simulink model "ferreira_charlton"  (R2024b)
settings: Solver=ode4  StartTime=0.0  StopTime=20  FixedStep=2e-4  RelTol=1e-3
InitFcn:
  | parameters_charlton;
  | parameters_ferreira;
  | KT = 1.44; Tmax = KT*Tmax;
  | Emax = 1.4;
  | LAP = 8.50;
undefined symbols (not defined in the file): AP_0, C3, Emin, Ferreira_LV, L, MCL_vascular_lib, P_venous, R1, R2, R3, R4, tc, V0, z1_0
settings Model: Creator=sammy  LastModifiedBy=sammy

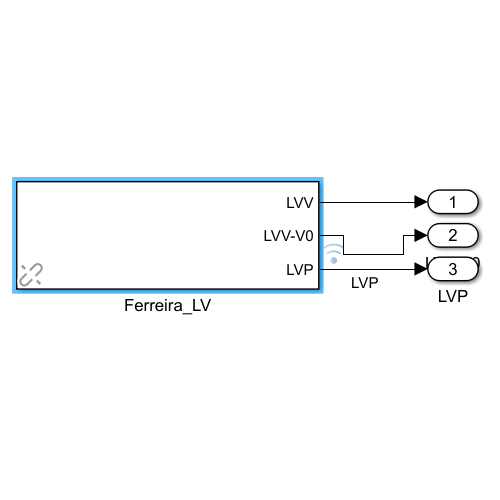
[thumbnail: Simulink's stored preview of the top-level diagram]
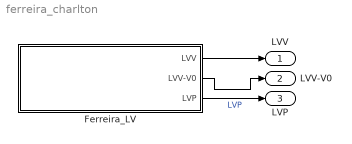
== system ferreira_charlton ==
  Ferreira_LV : Subsystem  AncestorBlock=MCL_vascular_lib/Ferreira_LV
  LVV : Outport
  LVV-V0 : Outport  Port=2
  LVP : Outport  Port=3
  wires:
  Ferreira_LV/3(LVP) -> LVP/1  "LVP"
  Ferreira_LV/2(LVV-V0) -> LVV-V0/1
  Ferreira_LV/1(LVV) -> LVV/1

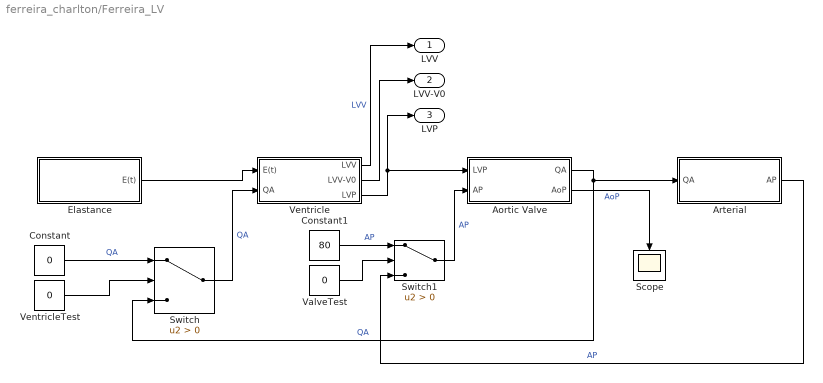
== system ferreira_charlton/Ferreira_LV ==
  Aortic Valve : Subsystem
  Arterial : Subsystem
  Constant : Constant  Value=0
  Constant1 : Constant  Value=80
  Elastance : Subsystem
  Scope : Scope
  Switch : Switch  Criteria=u2 > Threshold  SaturateOnIntegerOverflow=off  InputSameDT=off
  Switch1 : Switch  Criteria=u2 > Threshold  SaturateOnIntegerOverflow=off  InputSameDT=off
  ValveTest : Constant  Value=0
  Ventricle : Subsystem
  VentricleTest : Constant  Value=0
  LVV : Outport
  LVV-V0 : Outport  Port=2
  LVP : Outport  Port=3
  wires:
  VentricleTest/1 -> Switch/2
  Aortic Valve/1(QA) -> Arterial/1(QA), Switch/3  "QA"
  Ventricle/2(LVV-V0) -> LVV-V0/1
  Elastance/1(E(t)) -> Ventricle/1(E(t))
  Constant/1 -> Switch/1  "QA"
  Constant1/1 -> Switch1/1  "AP"
  Ventricle/3(LVP) -> LVP/1, Aortic Valve/1(LVP)
  Arterial/1(AP) -> Switch1/3  "AP"
  Switch/1 -> Ventricle/2(QA)  "QA"
  ValveTest/1 -> Switch1/2
  Switch1/1 -> Aortic Valve/2(AP)  "AP"
  Ventricle/1(LVV) -> LVV/1  "LVV"
  Aortic Valve/2(AoP) -> Scope/1  "AoP"

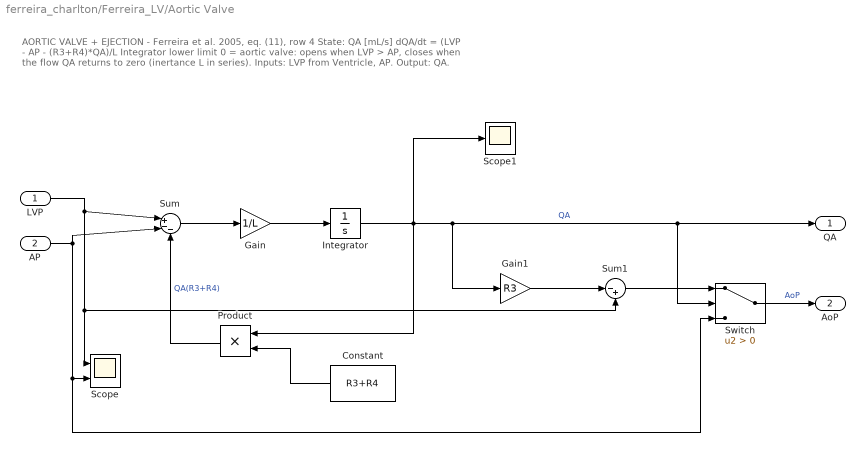
== system ferreira_charlton/Ferreira_LV/Aortic Valve ==
  note: AORTIC VALVE + EJECTION - Ferreira et al. 2005, eq. (11), row 4
      | State: QA [mL/s] dQA/dt = (LVP - AP - (R3+R4)*QA)/L
      | Integrator lower limit 0 = aortic valve: opens when LVP > AP, closes when the flow QA returns to zero (inertance L in series).
      | Inputs: LVP from Ventricle, AP. Output: QA.
  LVP : Inport
  AP : Inport  Port=2
  Constant : Constant  Value=R3+R4
  Gain : Gain  Gain=1/L
  Gain1 : Gain  Gain=R3
  Integrator : Integrator  LimitOutput=on  LowerSaturationLimit=0
  Product : Product
  Scope : Scope  NumInputPorts=2
  Scope1 : Scope
  Sum : Sum  Inputs=|+--
  Sum1 : Sum  Inputs=|-+
  Switch : Switch  Criteria=u2 > Threshold  SaturateOnIntegerOverflow=off  InputSameDT=off
  QA : Outport
  AoP : Outport  Port=2
  wires:
  LVP/1 -> Sum1/2, Scope/1, Sum/1
  AP/1 -> Switch/3, Scope/2, Sum/2
  Integrator/1 -> Scope1/1, Gain1/1, Switch/2, QA/1, Product/1  "QA"
  Constant/1 -> Product/2
  Product/1 -> Sum/3  "QA(R3+R4)"
  Sum/1 -> Gain/1
  Gain/1 -> Integrator/1
  Gain1/1 -> Sum1/1
  Sum1/1 -> Switch/1
  Switch/1 -> AoP/1  "AoP"

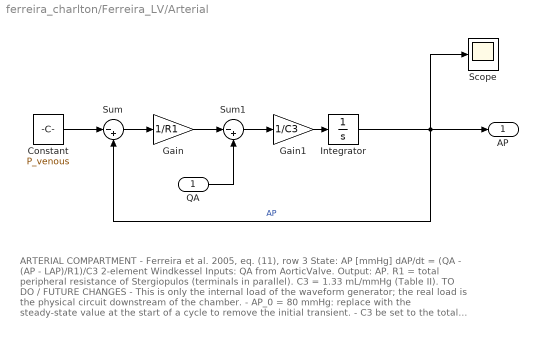
== system ferreira_charlton/Ferreira_LV/Arterial ==
  note: ARTERIAL COMPARTMENT - Ferreira et al. 2005, eq. (11), row 3
      | State: AP [mmHg] dAP/dt = (QA - (AP - LAP)/R1)/C3 2-element Windkessel
      | Inputs: QA from AorticValve. Output: AP. R1 = total peripheral resistance of Stergiopulos (terminals in parallel). C3 = 1.33 mL/mmHg (Table II).
      | TO DO / FUTURE CHANGES
      | - This is only the internal load of the waveform generator; the real load is the physical circuit downstream of the chamber.
      | - AP_0 = 80 mmHg: replace with the steady-state value at the start of a cycle to remove the initial transient.
      | - C3 be set to the total compliance of the Stergiopulos model for consistency with R1
  QA : Inport
  Constant : Constant  Value=P_venous
  Gain : Gain  Gain=1/R1
  Gain1 : Gain  Gain=1/C3
  Integrator : Integrator  InitialCondition=AP_0
  Scope : Scope
  Sum : Sum  Inputs=|-+
  Sum1 : Sum  Inputs=|-+
  AP : Outport
  wires:
  Constant/1 -> Sum/1
  Integrator/1 -> Scope/1, AP/1, Sum/2  "AP"
  Sum/1 -> Gain/1
  Gain/1 -> Sum1/1
  QA/1 -> Sum1/2
  Sum1/1 -> Gain1/1
  Gain1/1 -> Integrator/1

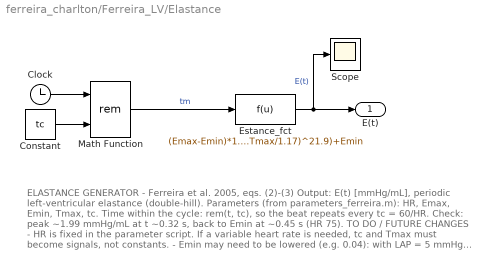
== system ferreira_charlton/Ferreira_LV/Elastance ==
  note: ELASTANCE GENERATOR - Ferreira et al. 2005, eqs. (2)-(3)
      | Output: E(t) [mmHg/mL], periodic left-ventricular elastance (double-hill).
      | Parameters (from parameters_ferreira.m):
      | HR, Emax, Emin, Tmax, tc.
      | Time within the cycle: rem(t, tc), so the beat repeats every tc = 60/HR.
      | Check: peak ~1.99 mmHg/mL at t ~0.32 s, back to Emin at ~0.45 s (HR 75).
      | TO DO / FUTURE CHANGES
      | - HR is fixed in the parameter script. If a variable heart rate is needed, tc and Tmax must become signals, not constants.
      | - Emin may need to be lowered (e.g. 0.04): with LAP = 5 mmHg the ventricle fills only to z1 = LAP/Emin ~ 83 mL (low stroke volume).
  Clock : Clock
  Constant : Constant  Value=tc
  Estance_fct : Fcn  Expr=(Emax-Emin)*1.55*((u/Tmax/0.7)^1.9/(1+(u/Tmax/0.7)^1.9))/(1+(u/Tmax/1.17)^21.9)+Emin
  Math Function : Math  Operator=rem
  Scope : Scope
  E(t) : Outport
  wires:
  Clock/1 -> Math Function/1
  Math Function/1 -> Estance_fct/1  "tm"
  Constant/1 -> Math Function/2
  Estance_fct/1 -> Scope/1, E(t)/1  "E(t)"

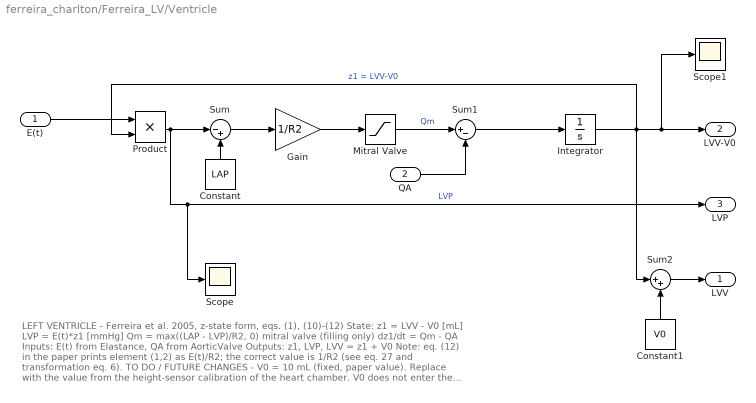
== system ferreira_charlton/Ferreira_LV/Ventricle ==
  note: LEFT VENTRICLE - Ferreira et al. 2005, z-state form, eqs. (1), (10)-(12)
      | State: z1 = LVV - V0 [mL] LVP = E(t)*z1 [mmHg] Qm = max((LAP - LVP)/R2, 0) mitral valve (filling only) dz1/dt = Qm - QA
      | Inputs: E(t) from Elastance, QA from AorticValve
      | Outputs: z1, LVP, LVV = z1 + V0
      | Note: eq. (12) in the paper prints element (1,2) as E(t)/R2; the correct value is 1/R2 (see eq. 27 and transformation eq. 6).
      | TO DO / FUTURE CHANGES
      | - V0 = 10 mL (fixed, paper value). Replace with the value from the height-sensor calibration of the heart chamber. V0 does not enter the dynamics, only the output LVV = z1 + V0. - LAP = P_venous (5 mmHg, constant), taken from parameters_stergiopulos.m. . - The output used by the physical chamber is the volume (LVV or z1); the conversion to pressure / chamber command is done outside this block.
  E(t) : Inport
  QA : Inport  Port=2
  Constant : Constant  Value=LAP
  Constant1 : Constant  Value=V0
  Gain : Gain  Gain=1/R2
  Integrator : Integrator  InitialCondition=z1_0
  Mitral Valve : Saturate  UpperLimit=inf  LowerLimit=0
  Product : Product
  Scope : Scope
  Scope1 : Scope
  Sum : Sum  Inputs=|-+
  Sum1 : Sum  Inputs=|+-
  Sum2 : Sum  Inputs=|++
  LVV : Outport
  LVV-V0 : Outport  Port=2
  LVP : Outport  Port=3
  wires:
  E(t)/1 -> Product/1
  Integrator/1 -> Sum2/1, Scope1/1, LVV-V0/1, Product/2  "z1 = LVV-V0"
  Product/1 -> Scope/1, LVP/1, Sum/1  "LVP"
  Constant/1 -> Sum/2
  Sum/1 -> Gain/1
  Gain/1 -> Mitral Valve/1
  Mitral Valve/1 -> Sum1/1  "Qm"
  QA/1 -> Sum1/2
  Sum1/1 -> Integrator/1
  Constant1/1 -> Sum2/2
  Sum2/1 -> LVV/1
